simulink model "SafeBeat_v1_step12_test"  (R2019a)
settings: Solver=FixedStepDiscrete  StartTime=0.0  StopTime=10.0  FixedStep=0.01  RelTol=1e-3
libraries: simulink x5, dsparch4 x1
settings Model: Creator=Admin  LastModifiedBy=Admin

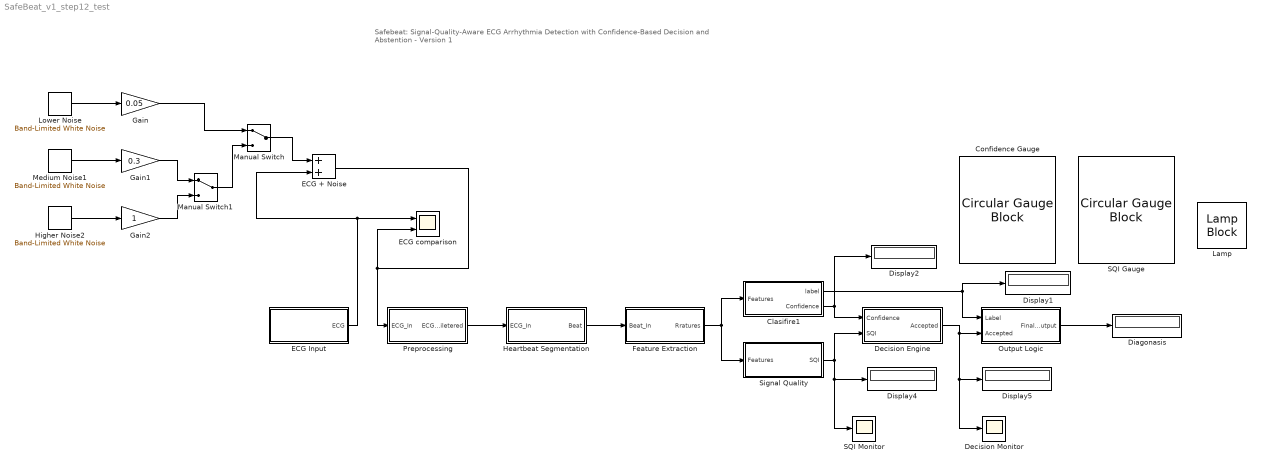
== system SafeBeat_v1_step12_test ==
  note: Safebeat: Signal-Quality-Aware ECG Arrhythmia Detection with Confidence-Based Decision and Abstention - Version 1
  Clasifire1 : Subsystem
  Confidence Gauge : CircularGaugeBlock  ScaleMax=1
  Decision Engine : Subsystem
  Decision Monitor : Scope
  "Diagonasis " : Display
  Display{1..2,4..5} (4 alike) : Display
  ECG + Noise : Sum
  ECG Input : Subsystem
  ECG comparison : Scope  NumInputPorts=2
  Feature Extraction : Subsystem
  Gain : Gain  Gain=0.05
  Gain1 : Gain  Gain=0.3
  Gain2 : Gain
  Heartbeat Segmentation : Subsystem
  Higher Noise2 : simulink/Sources/Band-Limited White Noise  Cov=1  Ts=0.01  seed=9999
  Lamp : LampBlock
  Lower Noise : simulink/Sources/Band-Limited White Noise  Cov=1  Ts=0.01  seed=1234
  Manual Switch : ManualSwitch
  Manual Switch1 : ManualSwitch
  Medium Noise1 : simulink/Sources/Band-Limited White Noise  Cov=1  Ts=0.01  seed=5678
  Output Logic : Subsystem
  Preprocessing : Subsystem
  SQI Gauge : CircularGaugeBlock  ScaleMax=1
  SQI Monitor : Scope
  Signal Quality : Subsystem
  wires:
  Preprocessing/1(ECG_Filetered) -> Heartbeat Segmentation/1(ECG_In)
  Heartbeat Segmentation/1("Beat ") -> Feature Extraction/1(Beat_In)
  Feature Extraction/1(Rratures) -> Clasifire1/1(Features), Signal Quality/1(Features)
  Clasifire1/2(Confidence) -> Display2/1, Decision Engine/1(Confidence)
  Clasifire1/1(label) -> Display1/1, Output Logic/1(Label)
  Signal Quality/1(SQI) -> Decision Engine/2(SQI), SQI Monitor/1, Display4/1
  Decision Engine/1(Accepted) -> Output Logic/2(Accepted), Decision Monitor/1, Display5/1
  Output Logic/1(FinalOutput) -> "Diagonasis "/1
  Lower Noise/1 -> Gain/1
  Medium Noise1/1 -> Gain1/1
  Higher Noise2/1 -> Gain2/1
  ECG Input/1(ECG) -> ECG comparison/1, ECG + Noise/2
  Manual Switch/1 -> ECG + Noise/1
  Gain/1 -> Manual Switch/1
  Gain1/1 -> Manual Switch1/1
  Gain2/1 -> Manual Switch1/2
  Manual Switch1/1 -> Manual Switch/2
  ECG + Noise/1 -> ECG comparison/2, Preprocessing/1(ECG_In)

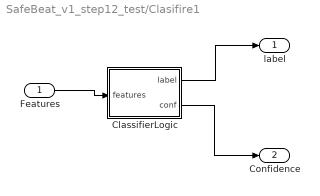
== system SafeBeat_v1_step12_test/Clasifire1 ==
  Features : Inport
  ClassifierLogic : MATLAB Function  TreatAsAtomicUnit=on
  label : Outport
  Confidence : Outport  Port=2
  wires:
  ClassifierLogic/1(label) -> label/1
  Features/1 -> ClassifierLogic/1(features)
  ClassifierLogic/2(conf) -> Confidence/1

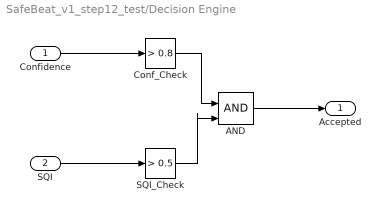
== system SafeBeat_v1_step12_test/Decision Engine ==
  Confidence : Inport
  SQI : Inport  Port=2
  AND : Logic  IconShape=distinctive  AllPortsSameDT=off  OutDataTypeStr=boolean
  Conf_Check : simulink/Logic and Bit Operations/Compare To Constant  relop=>  const=0.8  OutDataTypeStr=boolean
  SQI_Check : simulink/Logic and Bit Operations/Compare To Constant  relop=>  const=0.5  OutDataTypeStr=boolean
  Accepted : Outport
  wires:
  Confidence/1 -> Conf_Check/1
  Conf_Check/1 -> AND/1
  SQI/1 -> SQI_Check/1
  SQI_Check/1 -> AND/2
  AND/1 -> Accepted/1

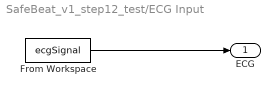
== system SafeBeat_v1_step12_test/ECG Input ==
  "From Workspace " : FromWorkspace  VariableName=ecgSignal  SampleTime=0
  ECG : Outport
  wires:
  "From Workspace "/1 -> ECG/1

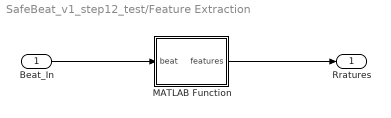
== system SafeBeat_v1_step12_test/Feature Extraction ==
  Beat_In : Inport
  MATLAB Function : MATLAB Function  TreatAsAtomicUnit=on
  Rratures : Outport
  wires:
  MATLAB Function/1(features) -> Rratures/1
  Beat_In/1 -> MATLAB Function/1(beat)

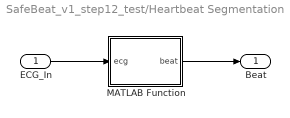
== system SafeBeat_v1_step12_test/Heartbeat Segmentation ==
  ECG_In : Inport
  MATLAB Function : MATLAB Function  TreatAsAtomicUnit=on
  "Beat " : Outport
  wires:
  ECG_In/1 -> MATLAB Function/1(ecg)
  MATLAB Function/1(beat) -> "Beat "/1

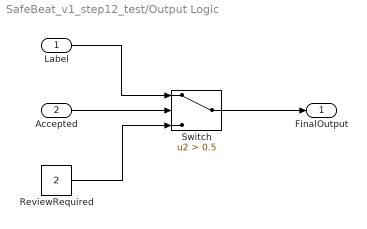
== system SafeBeat_v1_step12_test/Output Logic ==
  Label : Inport
  Accepted : Inport  Port=2
  ReviewRequired : Constant  Value=2
  Switch : Switch  Criteria=u2 > Threshold  Threshold=0.5
  FinalOutput : Outport
  wires:
  Switch/1 -> FinalOutput/1
  Label/1 -> Switch/1
  Accepted/1 -> Switch/2
  ReviewRequired/1 -> Switch/3

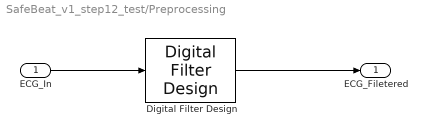
== system SafeBeat_v1_step12_test/Preprocessing ==
  ECG_In : Inport
  Digital Filter Design : dsparch4/Digital Filter Design  mwdsp_browser_bugfix_var=off
  ECG_Filetered : Outport
  wires:
  ECG_In/1 -> Digital Filter Design/1
  Digital Filter Design/1 -> ECG_Filetered/1

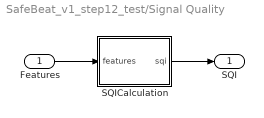
== system SafeBeat_v1_step12_test/Signal Quality ==
  Features : Inport
  SQICalculation : MATLAB Function  TreatAsAtomicUnit=on
  SQI : Outport
  wires:
  Features/1 -> SQICalculation/1(features)
  SQICalculation/1(sqi) -> SQI/1

== matlab function SafeBeat_v1_step12_test/Feature Extraction/MATLAB Function ==
  data: beat input; features output size=[4 1]
function features = fcn(beat)

meanVal = mean(beat);

stdVal = std(beat);

energyVal = sum(beat.^2);

peakVal = max(abs(beat));

features = [
    meanVal;
    stdVal;
    energyVal;
    peakVal
];

end

== matlab function SafeBeat_v1_step12_test/Heartbeat Segmentation/MATLAB Function ==
  data: ecg input; beat output size=[250 1]
function beat = fcn(ecg)

persistent buffer

if isempty(buffer)
    buffer = zeros(250,1);
end

buffer = [buffer(2:end); ecg];

beat = buffer;

== matlab function SafeBeat_v1_step12_test/Signal Quality/SQICalculation ==
  data: features input; sqi output double size=1
function sqi = calcSQI(features)

noiseMetric = features(2);

sqi = 1/(1 + noiseMetric);

end

== matlab function SafeBeat_v1_step12_test/Clasifire1/ClassifierLogic ==
  data: features input; label output double size=1; conf output double size=1
function [label, conf] = classify(features)

energy = features(3);

if energy > 100

    label = 1;
    conf = 0.90;

else

    label = 0;
    conf = 0.85;

end

end
